simulink model "Selector_Consigna"  (R2026b)
settings: Solver=VariableStepAuto
values from neighbouring files (symbols this model uses):
  r = 120.0    (= 120)    [coeficientes.m]
settings Model: Creator=fedeb  LastModifiedBy=fedeb

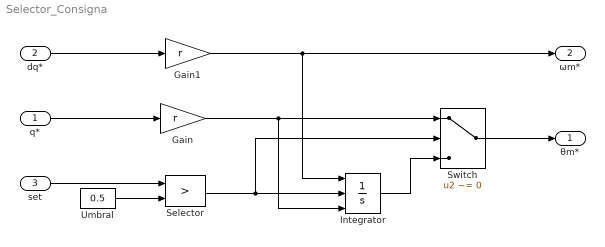
== system Selector_Consigna ==
  q* : Inport
  dq* : Inport  Port=2
  set : Inport  Port=3
  Gain : Gain  Gain=r
  Gain1 : Gain  Gain=r
  Integrator : Integrator  ExternalReset=level  InitialConditionSource=external
  Selector : RelationalOperator  Operator=>  OutDataTypeStr=boolean  RndMeth=Simplest  InputSameDT=off
  Switch : Switch  Criteria=u2 ~= 0  SaturateOnIntegerOverflow=off  InputSameDT=off
  Umbral : Constant  Value=0.5
  θm* : Outport
  ωm* : Outport  Port=2
  wires:
  q*/1 -> Gain/1
  dq*/1 -> Gain1/1
  set/1 -> Selector/1
  Umbral/1 -> Selector/2
  Gain/1 -> Switch/1, Integrator/3
  Selector/1 -> Switch/2, Integrator/2
  Gain1/1 -> ωm*/1, Integrator/1
  Integrator/1 -> Switch/3
  Switch/1 -> θm*/1
